simulink model "sfGetStartedLogging"  (R2025b)
settings: Solver=VariableStepAuto  StartTime=0.0  StopTime=10.0  RelTol=1e-3
settings Model: Creator=The MathWorks, Inc.  LastModifiedBy=The MathWorks, Inc.

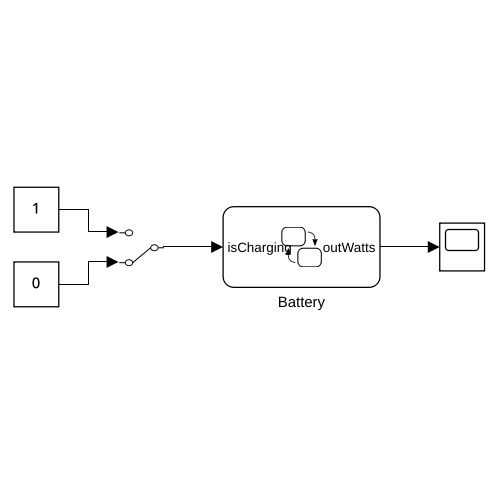
[thumbnail: Simulink's stored preview of the top-level diagram]
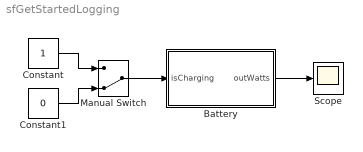
== system sfGetStartedLogging ==
  Battery : Stateflow chart  TreatAsAtomicUnit=on
  Constant : Constant
  Constant1 : Constant  Value=0
  Manual Switch : ManualSwitch  CurrentSetting=0
  Scope : Scope
      settings: ActiveDisplayYMinimum=-0.43749999999999989  ActiveDisplayYMaximum=3.9375
  wires:
  Manual Switch/1 -> Battery/1(isCharging)
  Constant/1 -> Manual Switch/1
  Constant1/1 -> Manual Switch/2
  Battery/1(outWatts) -> Scope/1

== stateflow chart sfGetStartedLogging/Battery ==
  state Charge
    entry:
    outWatts=0;
    during:
    chargePct=chargePct+4;
  state Discharge
    entry:
    outWatts=3.5;
    during:
    chargePct=chargePct-3;
  (default) -> Charge
  Charge -> Discharge : [~isCharging]
  Discharge -> Charge : [isCharging]
  data: isCharging input; outWatts output; chargePct local =50
